simulink subsystem "Day2_Scenario_4_5"  (R2024a)
settings: Solver=VariableStepAuto  StartTime=0.0  StopTime=10.0  RelTol=1e-3
undefined symbols (not defined in the file): route1_waypoint_raw
libraries: CarMaker4SL x6, slpidlib x1
settings Model: Creator=junhyung.cha  LastModifiedBy=junhyung.cha

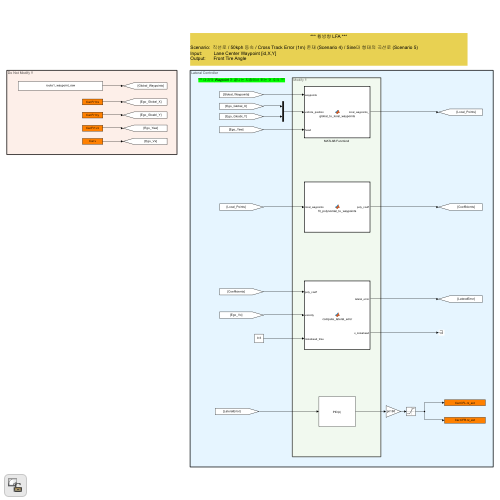
[thumbnail: Simulink's stored preview of the top-level diagram]
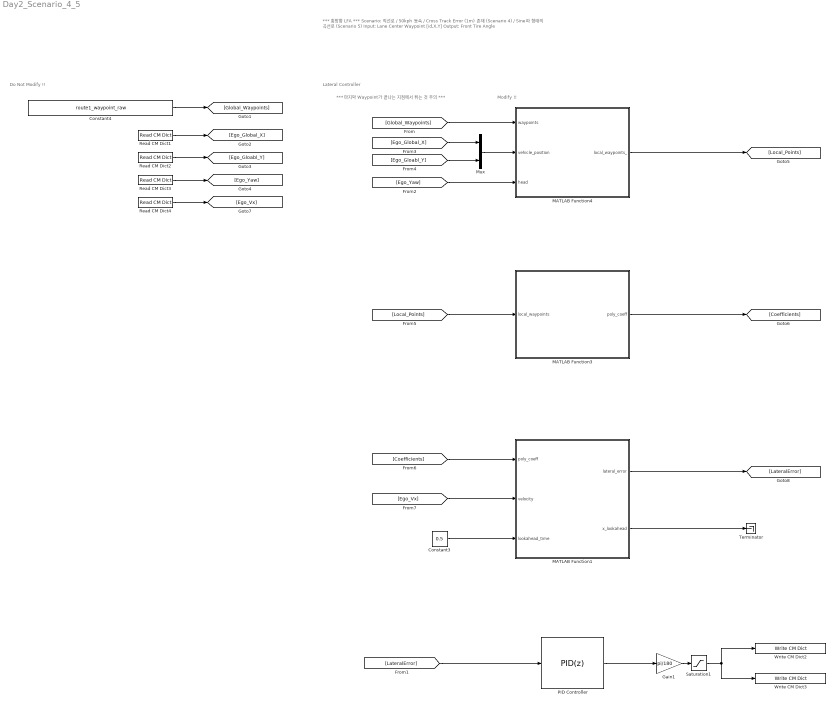
== system Day2_Scenario_4_5 ==
  note: *** 마지막 Waypoint가 끝나는 지점에서 튀는 것 주의 ***
  note: Modify !!
  note: Lateral Controller
  note: Do Not Modify !!
  note: *** 횡방향 LFA ***
      |
      | Scenario: 직선로 / 50kph 등속 / Cross Track Error (1m) 존재 (Scenario 4) / Sine파 형태의 곡선로 (Scenario 5)
      | Input: Lane Center Waypoint [id,X,Y]
      | Output: Front Tire Angle
  Constant3 : Constant  Value=0.5
  Constant4 : Constant  Value=route1_waypoint_raw
  Gain1 : Gain  Gain=pi/180
  MATLAB Function1 : MATLAB Function  TreatAsAtomicUnit=on
  MATLAB Function3 : MATLAB Function  TreatAsAtomicUnit=on
  "MATLAB Function4 " : MATLAB Function  TreatAsAtomicUnit=on
  Mux : Mux  Inputs=2
  PID Controller : slpidlib/PID Controller  Controller=PID  Form=Parallel  TimeDomain=Discrete-time  UseExternalTs=off  SampleTime=-1  IntegratorMethod=Forward Euler  FilterMethod=Forward Euler  ControllerParametersSource=internal  P=3  I=0.01  UseKiTs=off  D=0  UseExternalDerivativeSource=off  N=100  UseFilter=on  TunerSelectOption=Transfer Function Based (PID Tuner App)  InitialConditionSource=internal  InitialConditionForIntegrator=0  InitialConditionForFilter=0  DifferentiatorICPrevScaledInput=0  ExternalReset=none  TrackingMode=off  Kt=1  LimitOutput=off  SatLimitsSource=internal  UpperSaturationLimit=inf  LowerSaturationLimit=-inf  LinearizeAsGain=on  AntiWindupMode=none  Kb=1  LimitIntegrator=off  UpperIntegratorSaturationLimit=inf  LowerIntegratorSaturationLimit=-inf  POutMin=[]  POutMax=[]  IOutMin=[]  IOutMax=[]  DOutMin=[]  DOutMax=[]  NOutMin=[]  NOutMax=[]  SumOutMin=[]  SumOutMax=[]  SaturationOutMin=[]  SaturationOutMax=[]  PParamMin=[]  PParamMax=[]  IParamMin=[]  IParamMax=[]  DParamMin=[]  DParamMax=[]  NParamMin=[]  NParamMax=[]  KbParamMin=[]  KbParamMax=[]  KtParamMin=[]  KtParamMax=[]  KbOutMin=[]  KbOutMax=[]  KtOutMin=[]  KtOutMax=[]  IntegratorOutMin=[]  IntegratorOutMax=[]  FilterOutMin=[]  FilterOutMax=[]  SumI1OutMin=[]  SumI1OutMax=[]  SumI2OutMin=[]  SumI2OutMax=[]  SumI3OutMin=[]  SumI3OutMax=[]  SumI4OutMin=[]  SumI4OutMax=[]  SumDOutMin=[]  SumDOutMax=[]  DifferentiatorOutMin=[]  DifferentiatorOutMax=[]  FilterDiffOutCoefMin=[]  FilterDiffOutCoefMax=[]  ReciprocalOutMin=[]  ReciprocalOutMax=[]  SumDenOutMin=[]  SumDenOutMax=[]  SumNumOutMin=[]  SumNumOutMax=[]  DivideOutMin=[]  DivideOutMax=[]  UdiffTsProdOutMin=[]  UdiffTsProdOutMax=[]  NTsProdOutMin=[]  NTsProdOutMax=[]  UintegralTsProdOutMin=[]  UintegralTsProdOutMax=[]  UngainTsProdOutMin=[]  UngainTsProdOutMax=[]  ClampingZeroOutDataTypeStr=Inherit: Inherit via back propagation  ClampingZeroOutMin=[]  ClampingZeroOutMax=[]  FilterDenConstantOutDataTypeStr=Inherit: Inherit via back propagation  FilterDenConstantOutMin=[]  FilterDenConstantOutMax=[]  PCopyOutDataTypeStr=Inherit: Inherit via back propagation  PCopyOutMin=[]  PCopyOutMax=[]  NCopyOutDataTypeStr=Inherit: Inherit via back propagation  NCopyOutMin=[]  NCopyOutMax=[]  IntegratorContinuousStateAttributes=''  IntegratorStateMustResolveToSignalObject=off  IntegratorRTWStateStorageClass=Auto  FilterContinuousStateAttributes=''  FilterStateMustResolveToSignalObject=off  FilterRTWStateStorageClass=Auto  ParallelPVariant=InternalParameters  IdealPVariant=Disabled  IVariant=InternalParameters  DVariant=InternalParameters  IntegratorVariant=Discrete  SatVariant=Disabled  AWVariant=Passthrough  PCopyVariant=Disabled  TRVariant=Disabled  FdbkBlocksVariant=Forward  IdealPFdbkVariant=Disabled  SatFdbkVariant=Disabled  DerivativeFilterVariant=ForwardEulerFilter  NVariant=InternalParameters  NCopyVariant=Disabled  FilterICVariant=InternalICsFilter  IntegratorICVariant=InternalICs  ExternalResetVariant=Disabled  TRSumVariant=Passthrough  SumFdbkVariant=Disabled  SumVariant=Sum_PID  TsampFilterVariant=InternalTs  TsampNgainVariant=Passthrough  TsampIntegralVariant=Disabled_SignalSpec  ExternalSaturationOutDataTypeStr=Inherit: Same as second input  DerivativeSourceVariant=ErrorSignal
  Read CM Dict1 : CarMaker4SL/Read CM Dict  xname=Car.Fr1.tx  xsync=off  xstime=Inherited
  Read CM Dict2 : CarMaker4SL/Read CM Dict  xname=Car.Fr1.ty  xsync=off  xstime=Inherited
  Read CM Dict3 : CarMaker4SL/Read CM Dict  xname=Car.Fr1.rz  xsync=off  xstime=Inherited
  Read CM Dict4 : CarMaker4SL/Read CM Dict  xname=Car.v  xsync=off  xstime=Inherited
  Saturation1 : Saturate  UpperLimit=2  LowerLimit=-2
  Terminator : Terminator
  Write CM Dict2 : CarMaker4SL/Write CM Dict  xname=Car.CFL.rz_ext  xsync=off
  Write CM Dict3 : CarMaker4SL/Write CM Dict  xname=Car.CFR.rz_ext  xsync=off
  wires:
  Read CM Dict1/1 -> [Ego_Global_X]
  Read CM Dict2/1 -> [Ego_Gloabl_Y]
  Read CM Dict3/1 -> [Ego_Yaw]
  [Ego_Yaw] -> "MATLAB Function4 "/3(head)
  [Ego_Global_X] -> Mux/1
  [Ego_Gloabl_Y] -> Mux/2
  "MATLAB Function4 "/1(local_waypoints_) -> [Local_Points]
  [Global_Waypoints] -> "MATLAB Function4 "/1(waypoints)
  [Local_Points] -> MATLAB Function3/1(local_waypoints)
  MATLAB Function3/1(poly_coeff) -> [Coefficients]
  [Coefficients] -> MATLAB Function1/1(poly_coeff)
  Constant3/1 -> MATLAB Function1/3(lookahead_time)
  Saturation1/1 -> Write CM Dict3/1, Write CM Dict2/1
  MATLAB Function1/1(lateral_error) -> [LateralError]
  [LateralError] -> PID Controller/1
  [Ego_Vx] -> MATLAB Function1/2(velocity)
  Constant4/1 -> [Global_Waypoints]
  PID Controller/1 -> Gain1/1
  Gain1/1 -> Saturation1/1
  Mux/1 -> "MATLAB Function4 "/2(vehicle_position)
  MATLAB Function1/2(x_lookahead) -> Terminator/1
  Read CM Dict4/1 -> [Ego_Vx]

== matlab function Day2_Scenario_4_5/MATLAB Function1 ==
  settings: updateMethod=DISCRETE  sampleTime=0.05
  data: poly_coeff input; lateral_error output; velocity input; lookahead_time input; x_lookahead output
function [lateral_error,x_lookahead] = compute_lateral_error(poly_coeff, velocity, lookahead_time)
    lateral_error = 0;
    x_lookahead = 0;
end

== matlab function Day2_Scenario_4_5/MATLAB Function3 ==
  settings: updateMethod=DISCRETE  sampleTime=0.05
  data: local_waypoints input; poly_coeff output
function poly_coeff = fit_polynomial_to_waypoints(local_waypoints)
    poly_coeff = 0;
end

== matlab function Day2_Scenario_4_5/MATLAB Function4  ==
  settings: updateMethod=DISCRETE  sampleTime=0.05
  data: waypoints input; local_waypoints_ output; vehicle_position input; head input
function local_waypoints_ = global_to_local_waypoints(waypoints, vehicle_position, head)
    local_waypoints_ = 0;
end
